simulink model "throttle_control_table"  (R2026a)
settings: Solver=VariableStepAuto
undefined symbols (not defined in the file or in its folder): constantsSTADPOLE
settings Model: Creator=Eric  LastModifiedBy=Eric

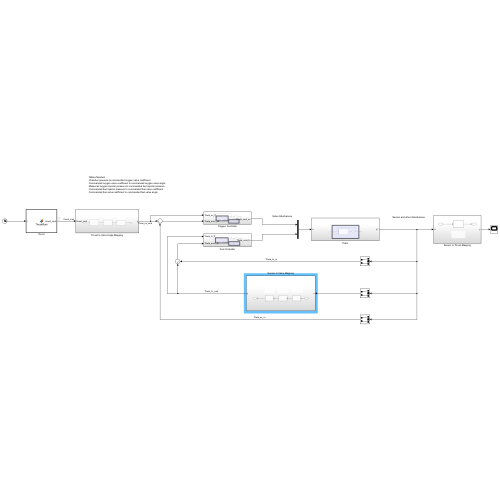
[thumbnail: Simulink's stored preview of the top-level diagram]
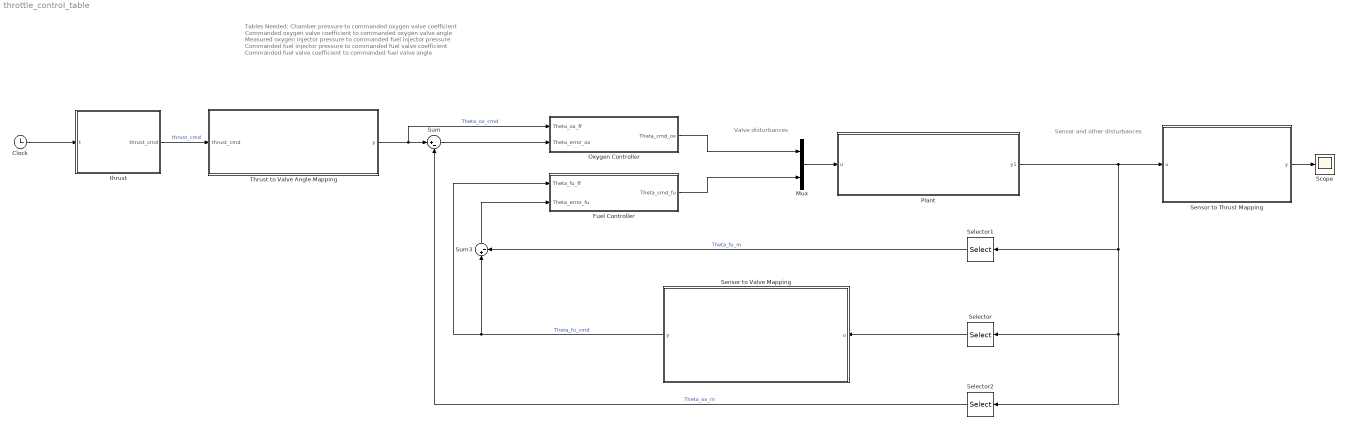
== system throttle_control_table ==
  note: Tables Needed:
      | Chamber pressure to commanded oxygen valve coefficient
      | Commanded oxygen valve coefficient to commanded oxygen valve angle
      | Measured oxygen injector pressure to commanded fuel injector pressure
      | Commanded fuel injector pressure to commanded fuel valve coefficient
      | Commanded fuel valve coefficient to commanded fuel valve angle
  note: Sensor and other disturbances
  note: Valve disturbances
  Clock : Clock
  Fuel Controller : Subsystem
  Mux : Mux  Inputs=2
  Oxygen Controller : Subsystem
  Plant : Subsystem
  Scope : Scope
  Selector : Selector  InputPortWidth=3  IndexOptions=Index vector (dialog)  Indices=[1 3]  OutputSizes=1
  Selector1 : Selector  InputPortWidth=3  IndexOptions=Index vector (dialog)  Indices=[1 3]  OutputSizes=1
  Selector2 : Selector  InputPortWidth=3  IndexOptions=Index vector (dialog)  Indices=[1 3]  OutputSizes=1
  Sensor to Thrust Mapping : Subsystem
  Sensor to Valve Mapping : Subsystem
  Sum : Sum  Inputs=|+-
  Sum3 : Sum  Inputs=|+-
  Thrust to Valve Angle Mapping : Subsystem
  thrust : MATLAB Function  TreatAsAtomicUnit=on
  wires:
  Clock/1 -> thrust/1(t)
  thrust/1(thrust_cmd) -> Thrust to Valve Angle Mapping/1(thrust_cmd)  "thrust_cmd"
  Thrust to Valve Angle Mapping/1(y) -> Oxygen Controller/1(Theta_ox_ff), Sum/1  "Theta_ox_cmd"
  Plant/1(y1) -> Selector2/1, Selector/1, Selector1/1, Sensor to Thrust Mapping/1(u)
  Sensor to Thrust Mapping/1(y) -> Scope/1
  Selector/1 -> Sensor to Valve Mapping/1(u)
  Selector2/1 -> Sum/2  "Theta_ox_m"
  Sensor to Valve Mapping/1(y) -> Sum3/1, Fuel Controller/1(Theta_fu_ff)  "Theta_fu_cmd"
  Selector1/1 -> Sum3/2  "Theta_fu_m"
  Sum/1 -> Oxygen Controller/2(Theta_error_ox)
  Sum3/1 -> Fuel Controller/2(Theta_error_fu)
  Fuel Controller/1(Theta_cmd_fu) -> Mux/2
  Mux/1 -> Plant/1(u)
  Oxygen Controller/1(Theta_cmd_ox) -> Mux/1

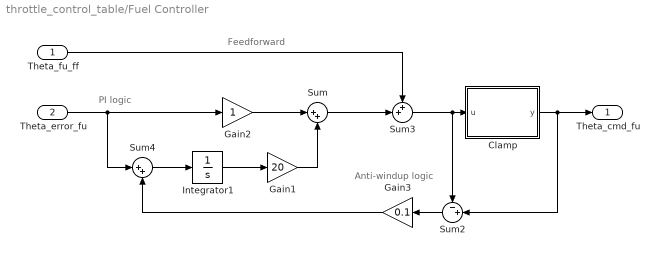
== system throttle_control_table/Fuel Controller ==
  note: Feedforward
  note: Anti-windup logic
  note: PI logic
  Theta_fu_ff : Inport
  Theta_error_fu : Inport  Port=2
  Clamp : MATLAB Function  TreatAsAtomicUnit=on
  Gain1 : Gain  Gain=20
  Gain2 : Gain
  Gain3 : Gain  Gain=0.1
  Integrator1 : Integrator
  Sum : Sum  Inputs=|++
  Sum2 : Sum  Inputs=-+|
  Sum3 : Sum  Inputs=++|
  Sum4 : Sum  Inputs=|++
  Theta_cmd_fu : Outport
  wires:
  Sum4/1 -> Integrator1/1
  Sum2/1 -> Gain3/1
  Sum3/1 -> Clamp/1(u), Sum2/1
  Clamp/1(y) -> Theta_cmd_fu/1, Sum2/2
  Theta_error_fu/1 -> Sum4/1, Gain2/1
  Theta_fu_ff/1 -> Sum3/1
  Integrator1/1 -> Gain1/1
  Gain2/1 -> Sum/1
  Gain1/1 -> Sum/2
  Sum/1 -> Sum3/2
  Gain3/1 -> Sum4/2

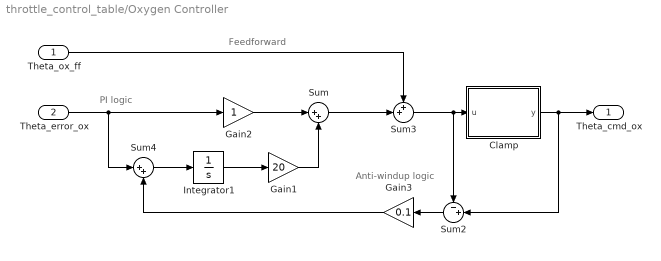
== system throttle_control_table/Oxygen Controller ==
  note: PI logic
  note: Anti-windup logic
  note: Feedforward
  Theta_ox_ff : Inport
  Theta_error_ox : Inport  Port=2
  Clamp : MATLAB Function  TreatAsAtomicUnit=on
  Gain1 : Gain  Gain=20
  Gain2 : Gain
  Gain3 : Gain  Gain=0.1
  Integrator1 : Integrator
  Sum : Sum  Inputs=|++
  Sum2 : Sum  Inputs=-+|
  Sum3 : Sum  Inputs=++|
  Sum4 : Sum  Inputs=|++
  Theta_cmd_ox : Outport
  wires:
  Sum3/1 -> Clamp/1(u), Sum2/1
  Clamp/1(y) -> Theta_cmd_ox/1, Sum2/2
  Theta_ox_ff/1 -> Sum3/1
  Sum2/1 -> Gain3/1
  Sum4/1 -> Integrator1/1
  Theta_error_ox/1 -> Sum4/1, Gain2/1
  Gain3/1 -> Sum4/2
  Gain1/1 -> Sum/2
  Gain2/1 -> Sum/1
  Sum/1 -> Sum3/2
  Integrator1/1 -> Gain1/1

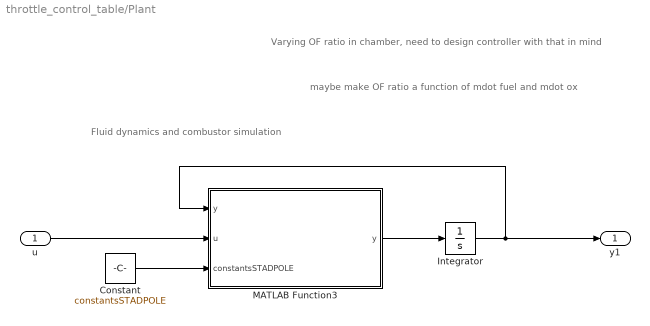
== system throttle_control_table/Plant ==
  note: Fluid dynamics and combustor simulation
  note: maybe make OF ratio a function of mdot fuel and mdot ox
  note: Varying OF ratio in chamber, need to design controller with that in mind
  u : Inport
  Constant : Constant  Value=constantsSTADPOLE  OutDataTypeStr=Bus: slBus1
  Integrator : Integrator  InitialCondition=constantsSTADPOLE.init_cond
  MATLAB Function3 : MATLAB Function  TreatAsAtomicUnit=on
  y1 : Outport
  wires:
  MATLAB Function3/1(y) -> Integrator/1
  Integrator/1 -> y1/1, MATLAB Function3/1("y ")
  Constant/1 -> MATLAB Function3/3(constantsSTADPOLE)
  u/1 -> MATLAB Function3/2(u)

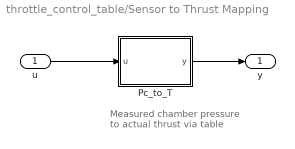
== system throttle_control_table/Sensor to Thrust Mapping ==
  note: Measured chamber pressure to actual thrust via table
  u : Inport
  Pc_to_T : MATLAB Function  TreatAsAtomicUnit=on
  y : Outport
  wires:
  Pc_to_T/1(y) -> y/1
  u/1 -> Pc_to_T/1(u)

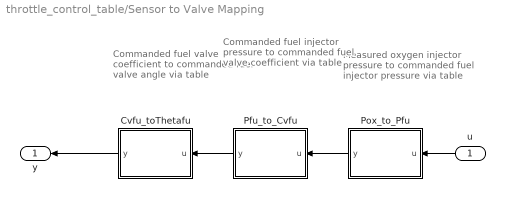
== system throttle_control_table/Sensor to Valve Mapping ==
  note: Measured oxygen injector pressure to commanded fuel injector pressure via table
  note: Commanded fuel valve coefficient to commanded fuel valve angle via table
  note: Commanded fuel injector pressure to commanded fuel valve coefficient via table
  u : Inport
  Cvfu_toThetafu : MATLAB Function  TreatAsAtomicUnit=on
  Pfu_to_Cvfu : MATLAB Function  TreatAsAtomicUnit=on
  Pox_to_Pfu : MATLAB Function  TreatAsAtomicUnit=on
  y : Outport
  wires:
  u/1 -> Pox_to_Pfu/1(u)
  Pfu_to_Cvfu/1(y) -> Cvfu_toThetafu/1(u)
  Cvfu_toThetafu/1(y) -> y/1
  Pox_to_Pfu/1(y) -> Pfu_to_Cvfu/1(u)

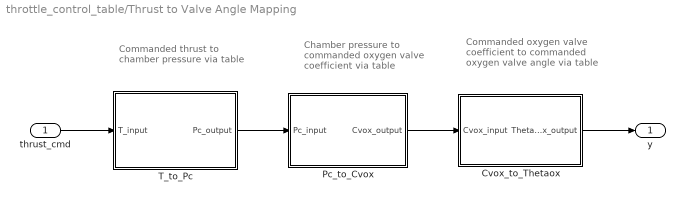
== system throttle_control_table/Thrust to Valve Angle Mapping ==
  note: Commanded oxygen valve coefficient to commanded oxygen valve angle via table
  note: Chamber pressure to commanded oxygen valve coefficient via table
  note: Commanded thrust to chamber pressure via table
  thrust_cmd : Inport
  Cvox_to_Thetaox : MATLAB Function  TreatAsAtomicUnit=on
  Pc_to_Cvox : MATLAB Function  TreatAsAtomicUnit=on
  T_to_Pc : MATLAB Function  TreatAsAtomicUnit=on
  y : Outport
  wires:
  Pc_to_Cvox/1(Cvox_output) -> Cvox_to_Thetaox/1(Cvox_input)
  T_to_Pc/1(Pc_output) -> Pc_to_Cvox/1(Pc_input)
  thrust_cmd/1 -> T_to_Pc/1(T_input)
  Cvox_to_Thetaox/1(Thetaox_output) -> y/1

== matlab function throttle_control_table/Thrust to Valve Angle Mapping/T_to_Pc ==
  data: T_input input; Pc_output output
function Pc_output = fcn(T_input)

table = readmatrix("[]", "NumHeaderLines", );
T_vector = table(:,1);
Pc_vector = table(:,2);

Pc_output = interp1(T_vector, Pc_vector, T_input);

== matlab function throttle_control_table/thrust ==
  data: t input; thrust_cmd output
function thrust_cmd = ThrustPlant(t)
% %THRUSTPLANT 
% %   random plant function for the thrust in the engine
% if t < 2
%     thrust_cmd = 0; %[N]
% elseif mod(t,5) < 3
%     thrust_cmd = 1500;
% else
%     thrust_cmd = 1500 - 500 * sin(mod(t,5) * pi / 2);
% 
% end
% %cosint(t*pi/180);
% 
% thrust_cmd = 1500;
if t < 3.0
    thrust_cmd = 2000; % [N] Step 1: 0s to 3s
elseif t < 6.0
    thrust_cmd = 1000; % [N] Step 2: 3s to 6s
else
    thrust_cmd = 1500;    % [N] Step 3: 6s to 10s
end

== matlab function throttle_control_table/Thrust to Valve Angle Mapping/Pc_to_Cvox ==
  data: Pc_input input; Cvox_output output
function Cvox_output = fcn(Pc_input)

table = readmatrix("[]", "NumHeaderLines", );
Pc_vector = table(:,1);
Cvox_vector = table(:,2);

Cvox_output = interp1(Pc_vector, Cvox_vector, Pc_input);

== matlab function throttle_control_table/Thrust to Valve Angle Mapping/Cvox_to_Thetaox ==
  data: Cvox_input input; Thetaox_output output
function Thetaox_output = fcn(Cvox_input)

table = readmatrix("[]", "NumHeaderLines", );
Cvox_vector = table(:,1);
Thetaox_vector = table(:,2);

Thetaox_output = interp1(Cvox_vector, Thetaox_vector, Cvox_input);

== matlab function throttle_control_table/Sensor to Valve Mapping/Cvfu_toThetafu ==
  data: u input; y output
function y = fcn(u)

y = u;

== matlab function throttle_control_table/Plant/MATLAB Function3 ==
  data: y input; u input; y output; constantsSTADPOLE input
function y = system_model(y, u, constantsSTADPOLE)
    
    % y(1)' = time rate of mass flow oxygen [kg/s^2]
    % y(2)' = time rate of mass flow fuel [kg/s^2]
    % y(3)' = time rate of chamber pressure [Pa/s]
    % y(4)' = time rate of oxygen injector press [Pa/s]
    % y(5)' = time rate of fuel injector press [Pa/s]
    % y(6)' = time rate of oxygen pressure at valve [Pa/s]
    % y(7)' = time rate of fuel pressure at valve [Pa/s]

    % y(1) = mass flow oxygen across pipe [kg/s]
    % y(2) = mass flow fuel across pipe [kg/s]
    % y(3) = chamber pressure [Pa]
    % y(4) = oxygen pressure at inj [Pa]
    % y(5) = fuel pressure at inj [Pa]
    % y(6) = oxygen pressure at valve [Pa]
    % y(7) = fuel pressure at valve [Pa]
    
    a_t= constantsSTADPOLE.a_t ; % [m^2], throat area
    
    dens_o = constantsSTADPOLE.dens_o; % [kg/m^3], liquid oxygen density, at 90 K and 1 atm
    dens_f = constantsSTADPOLE.dens_f ; % [kg/m^3], fuel density, at 293 K and 1 atm
    dens_w = constantsSTADPOLE.dens_w ; % [kg/m^3], water density
    g = constantsSTADPOLE.g ; % [m/s^2], acceleration due to gravity
    a_i_o = constantsSTADPOLE.a_i_o; % [m^2] area injector ox
    a_i_f = constantsSTADPOLE.a_i_f ; % [m^2] area injector fuel
    r = constantsSTADPOLE.r ; % [J/kg-K], specific gas constant of exhaust (molecular weight 18.8 g/mol)
    c_star = constantsSTADPOLE.c_star ; % [m/s] characteristic velocity
    of = constantsSTADPOLE.OF_target;

    c_fric = 0.03; % [unitless], line friction coefficient
    c_d_o = constantsSTADPOLE.d_coeff_ox; % [unitless], oxygen injector coefficient
    c_d_f = constantsSTADPOLE.d_coeff_fu; % [unitless], fuel injector coefficient
    l_eq_o = 7 * 0.0254; % [m], oxygen equivalent line length 
    l_eq_f = 7 * 0.0254; % [m], fuel equivalent line length 
    l_o = 120 * 0.0254; % [m], oxygen line length
    l_f = 60 * 0.0254; % [m], fuel line length
    d = (0.5 - 2 * 0.065) * 0.0254; % [m], line diameter
    v_c = 1.103170594 * 1e-3; % [m^3], chamber volume
    a_l = pi * (d / 2) ^ 2; % [m^2], line area
  
    v_l_o = a_l * l_o;
    v_l_f = a_l * l_f;
    t_o = 90; 
    t_f = 293;

    % Assume constant?
    c_v_o = u(1,1); %AngleToCoefficient(u(1,1));  % 1.231e-06; [m^3.5/kg^0.5], oxygen valve coefficient
    c_v_f = u(2,1); %AngleToCoefficient(u(2,1));  % 1.231e-06; [], fuel valve coefficient
    p_tank_o = 3.792E6; % [Pa]
    p_tank_f = 3.792E6; % [Pa]
    t_c = 3570; % [K], chamber temperature
    

    del_p_i_o = 1 / (2 * dens_o * (c_d_o * a_i_o) ^ 2); 
    del_p_l_o = 96402.2;
    del_p_i_f = 1 / (2 * dens_f * (c_d_f * a_i_f) ^ 2); 
    del_p_l_f = 2082581.1;
    

    % Momentum equations
    % massflow across pipe
    % mdot_pipe_ox = (y(4) - y(3) - del_p_l_o * y(1) * sqrt(y(1)^2 + 1e-6)) * a_l / l_o;
    % mdot_pipe_fu = (y(5) - y(3) - del_p_l_f * y(2) * sqrt(y(2)^2 + 1e-6)) * a_l / l_f;
    mddot_pipe_ox = (y(6) - y(4) - del_p_l_o * y(1) * sqrt(y(1)^2 + 1e-6)) * a_l / l_o;
    mddot_pipe_fu = (y(7) - y(5) - del_p_l_f * y(2) * sqrt(y(2)^2 + 1e-6)) * a_l / l_f;

    % Valve massflows
    ValveOX = dens_o * dens_w * (p_tank_o - y(6));
    ValveFU = dens_f * dens_w * (p_tank_f - y(7));
    mdot_valve_ox = c_v_o * ValveOX / sqrt(abs(ValveOX) + 1e2);
    mdot_valve_fu = c_v_f * ValveFU / sqrt(abs(ValveFU) + 1e2);

    % Injector massflows
    InjectorOX = 2 * dens_o *(y(4)-y(3));
    InjectorFU = 2 * dens_f * (y(5)-y(3));
    mdot_inj_ox = c_d_o * a_i_o * InjectorOX / sqrt(abs(InjectorOX)+1e2);
    mdot_inj_fu = c_d_f * a_i_f * InjectorFU / sqrt(abs(InjectorFU)+1e2);

    % Pressure at the end of the valve
    valve_ox_dot = 1e9 / (v_l_o * dens_o) * (mdot_valve_ox - y(1));
    valve_fu_dot = 1e9 / (v_l_f * dens_f) * (mdot_valve_fu - y(2));

    inj_ox_dot = 1e9 / (v_l_o*dens_o) * (y(1) - mdot_inj_ox);
    inj_fu_dot = 1e9 / (v_l_f*dens_f) * (y(2) - mdot_inj_fu);

    % Chamber Pressure equations
    pdot_chamber = (r * t_c / v_c) * (mdot_inj_ox + mdot_inj_fu - a_t * y(3) / c_star);

    % Final system
    y = [mddot_pipe_ox; mddot_pipe_fu; pdot_chamber; inj_ox_dot; inj_fu_dot; valve_ox_dot; valve_fu_dot];
end

== matlab function throttle_control_table/Sensor to Valve Mapping/Pfu_to_Cvfu ==
  data: u input; y output
function y = fcn(u)

y = u;

== matlab function throttle_control_table/Sensor to Valve Mapping/Pox_to_Pfu ==
  data: u input; y output
function y = fcn(u)

y = u;

== matlab function throttle_control_table/Oxygen Controller/Clamp ==
  data: u input; y output
function y = sat(u)

if u < 0
    y = 0;

elseif 90 < u
    y = 90;

else
    y = u;

end

== matlab function throttle_control_table/Sensor to Thrust Mapping/Pc_to_T ==
  data: u input; y output
function y = fcn(u)

y = u;

== matlab function throttle_control_table/Fuel Controller/Clamp ==
  data: u input; y output
function y = sat(u)

if u < 0
    y = 0;

elseif 90 < u
    y = 90;

else
    y = u;

end
